simulink model "TVC_Hover_Plant_Coaxial_Articulated"  (R2025b)
settings: Solver=ode45  StartTime=0.0  StopTime=12  MaxStep=0.02  RelTol=1e-6
model workspace (MAT data in the model file):
  Sig = Simulink.Signal
  Sig.Dimensions = -1
  Sig.DimensionsMode = 'auto'
  Sig.Complexity = 'auto'
  Sig.SampleTime = -1
  Sig.SamplingMode = 'auto'
  Sig.DataType = 'auto'
  Sig1 = Simulink.Signal
  Sig1.Dimensions = -1
  Sig1.DimensionsMode = 'auto'
  Sig1.Complexity = 'auto'
  Sig1.SampleTime = -1
  Sig1.SamplingMode = 'auto'
  Sig1.DataType = 'auto'
  Sig2 = Simulink.Signal
  Sig2.Dimensions = -1
  Sig2.DimensionsMode = 'auto'
  Sig2.Complexity = 'auto'
  Sig2.SampleTime = -1
  Sig2.SamplingMode = 'auto'
  Sig2.DataType = 'auto'
  Sig3 = Simulink.Signal
  Sig3.Dimensions = -1
  Sig3.DimensionsMode = 'auto'
  Sig3.Complexity = 'auto'
  Sig3.SampleTime = -1
  Sig3.SamplingMode = 'auto'
  Sig3.DataType = 'auto'
  Sig4 = Simulink.Signal
  Sig4.Dimensions = -1
  Sig4.DimensionsMode = 'auto'
  Sig4.Complexity = 'auto'
  Sig4.SampleTime = -1
  Sig4.SamplingMode = 'auto'
  Sig4.DataType = 'auto'
  Sig5 = Simulink.Signal
  Sig5.Dimensions = -1
  Sig5.DimensionsMode = 'auto'
  Sig5.Complexity = 'auto'
  Sig5.SampleTime = -1
  Sig5.SamplingMode = 'auto'
  Sig5.DataType = 'auto'
  TVC_ARTICULATION_ENABLED = 1
  TVC_FAN1_KQ = 0.012
  TVC_FAN2_KQ = 0.012
  TVC_FAN_CG_OFFSET_M = [0; 0; 0]
  TVC_GRAVITY_MPS2 = 9.80665
  TVC_INERTIA_KGM2 = [0.003  0  0; 0  0.016  0; 0  0  0.016]
  TVC_I_FAN_CG_KGM2 = [0  0  0; 0  0  0; 0  0  0]
  TVC_I_UPPER_CG_KGM2 = [0.00105  0  0; 0  0.0056  0; 0  0  0.0056]
  TVC_JOINT_DIFF_TAU_S = 0.02
  TVC_JOINT_DIFF_TS_S = 0.01
  TVC_LINK1_M = [-0.084; 0; 0]
  TVC_LINK2_M = [-0.097; 0; 0]
  TVC_MASS_FAN_KG = 0.224
  TVC_MASS_KG = 0.8
  TVC_MASS_LINK1_KG = 0.264
  TVC_MASS_LINK2_KG = 0.248
  TVC_MASS_UPPER_KG = 0.464
  TVC_PIVOT_B_M = [-0.12; 0; 0]
  TVC_SERVO_MAX_DEG = 20
  TVC_TMAX1_N = 8
  TVC_TMAX2_N = 8
settings Model: Creator=shhan  LastModifiedBy=shhan

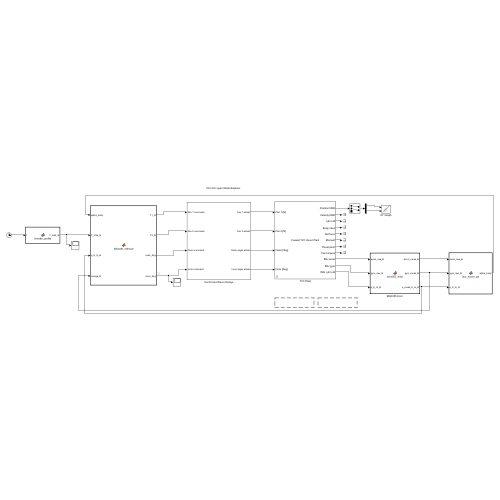
[thumbnail: Simulink's stored preview of the top-level diagram]
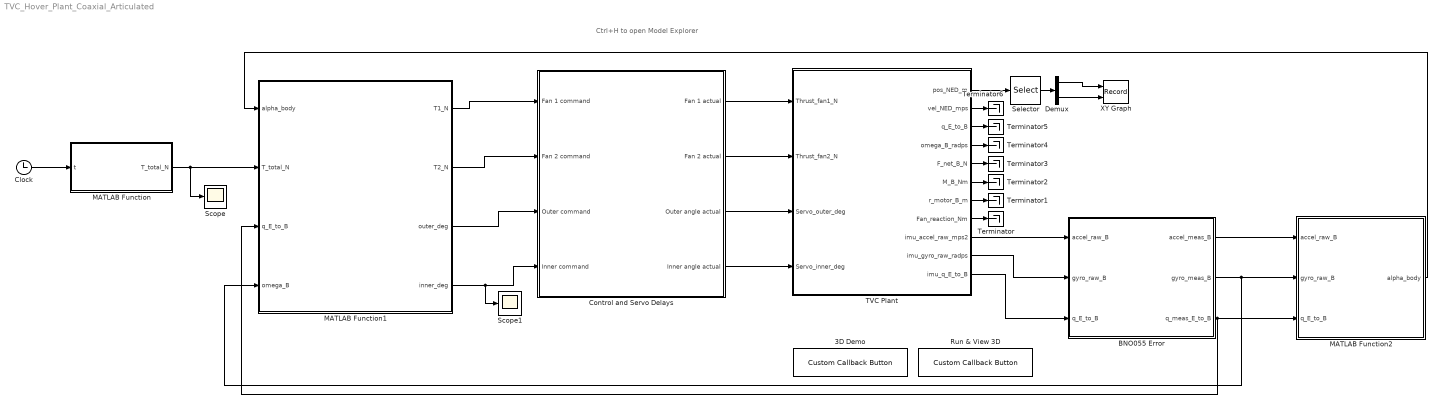
== system TVC_Hover_Plant_Coaxial_Articulated ==
  note: Ctrl+H to open Model Explorer
  3D Demo : CustomCallbackButton  Tag=TVCReplayButton  Configuration="{\"components\":[{\"name\":\"BackgroundImageComponent\",\"settings\":{\"image\":{\"size\":[0,0],\"src\":\"default\",\"srcOrientation\":\"Right\"},\"position\":[0,0,1,1]}},{\"name\":\"ButtonStateComponent\",\"settings\":{\"buttonType\":\"momentary\",\"clickFcn\":\"build_TVC_hover_plant('diagram-demo', bdroot());\",\"onValue\":1,\"position\":[0,0,1,1],\"pressDelay\":\"500\",\"pressFcn\":\"\",\"repeatInterval\":\"0\",\"states\":[{\"horizontalAlignment\":\"center\",\"image\":{\"position\":[0,0,1,1],\"size\":[1,1],\"src\":\"default\",\"srcOrientation\":\"Right\"},\"label\":{\"color\":[0.01176470588,0.01176470588,0.01176470588,1],\"icon\":{\"size\":[0,0],\"src\":\"default\",\"srcOrientation\":\"Right\"},\"iconOffset\":0,\"iconPlacement\":\"left\",\"opacity\":1,\"show\":true,\"text\":{\"content\":\"3D Demo\",\"font\":\"Helvetica\"}},\"labelOffset\":[0,0],\"verticalAlignment\":\"middle\"},{\"horizontalAlignment\":\"center\",\"image\":{\"position\":[0,0,1,1],\"size\":[1,1],\"src\":\"default\",\"srcOrientation\":\"Right\"},\"label\":{\"color\":[0.01176470588,0.01176470588,0.01176470588,1],\"icon\":{\"size\":[0,0],\"src\":\"default\",\"srcOrientation\":\"Right\"},\"iconOffset\":0,\"iconPlacement\":\"left\",\"opacity\":1,\"show\":true,\"text\":{\"content\":\"3D Demo\",\"font\":\"Helvetica\"}},\"labelOffset\":[0,0],\"verticalAlignment\":\"middle\"},{\"horizontalAlignment\":\"center\",\"image\":{\"position\":[0,0,1,1],\"size\":[1,1],\"src\":\"default\",\"srcOrientation\":\"Right\"},\"label\":{\"color\":[0.01176470588,0.01176470588,0.01176470588,1],\"icon\":{\"size\":[0,0],\"src\":\"default\",\"srcOrientation\":\"Right\"},\"iconOffset\":0,\"iconPlacement\":\"left\",\"opacity\":1,\"show\":true,\"text\":{\"content\":\"3D Demo\",\"font\":\"Helvetica\"}},\"labelOffset\":[0,0],\"verticalAlignment\":\"middle\"},{\"horizontalAlignment\":\"center\",\"image\":{\"position\":[0,0,1,1],\"size\":[1,1],\"src\":\"default\",\"srcOrientation\":\"Right\"},\"label\":{\"color\":[0.01176470588,0.01176470588,0.01176470588,1],\"icon\":{\"size\":[0,0],\"src\":\"default\",\"srcOrientation\":\"Right\"},\"iconOffset\":0,\"iconPlacement\":\"left\",\"opacity\":1,\"show\":true,\"text\":{\"content\":\"3D Demo\",\"font\":\"Helvetica\"}},\"labelOffset\":[0,0],\"verticalAlignment\":\"middle\"}]}},{\"name\":\"ForegroundImageComponent\",\"settings\":{\"image\":{\"size\":[0,0],\"src\":\"default\",\"srcOrientation\":\"Right\"},\"isForeground\":1,\"position\":[0,0,1,1]}}],\"derived\":{\"blockParameters\":{\"AutoActivate\":true,\"ButtonText\":\"3D Demo\",\"ButtonType\":\"Momentary\",\"ClickFcn\":\"build_TVC_hover_plant('diagram-demo', bdroot());\",\"OnValue\":1,\"PressDelay\":\"500\",\"PressFcn\":\"\",\"RepeatInterval\":\"0\",\"fixedAspectRatio\":\"off\"}},\"settings\":{\"BindingType\":\"standalone\",\"autoActivate\":true,\"backgroundColor\":[244,244,244,1],\"backgroundOffset\":0.2,\"backgroundOpacity\":1,\"fixedAspectRatio\":\"off\",\"foregroundColor\":[0.01176470588,0.01176470588,0.01176470588,1],\"migratedFromLegacy\":true,\"useBackgroundColor\":true,\"variant\":\"callback\",\"version\":\"R2025a\"},\"type\":\"Button\"}"  CustomBackgroundColor="{\"color\":[0.9568627451,0.9568627451,0.9568627451],\"show\":true}"
  BNO055 Error : MATLAB Function  TreatAsAtomicUnit=on
  Clock : Clock
  Control and Servo Delays : Subsystem  Tag=TVCControllerAndServoTiming
  Demux : Demux  Outputs=2
  MATLAB Function : MATLAB Function  TreatAsAtomicUnit=on
  MATLAB Function1 : MATLAB Function  TreatAsAtomicUnit=on
  MATLAB Function2 : MATLAB Function  TreatAsAtomicUnit=on
  Run & View 3D : CustomCallbackButton  Tag=TVCReplayButton  Configuration="{\"components\":[{\"name\":\"BackgroundImageComponent\",\"settings\":{\"image\":{\"size\":[0,0],\"src\":\"default\",\"srcOrientation\":\"Right\"},\"position\":[0,0,1,1]}},{\"name\":\"ButtonStateComponent\",\"settings\":{\"buttonType\":\"momentary\",\"clickFcn\":\"build_TVC_hover_plant('diagram-run', bdroot());\",\"onValue\":1,\"position\":[0,0,1,1],\"pressDelay\":\"500\",\"pressFcn\":\"\",\"repeatInterval\":\"0\",\"states\":[{\"horizontalAlignment\":\"center\",\"image\":{\"position\":[0,0,1,1],\"size\":[1,1],\"src\":\"default\",\"srcOrientation\":\"Right\"},\"label\":{\"color\":[0.01176470588,0.01176470588,0.01176470588,1],\"icon\":{\"size\":[0,0],\"src\":\"default\",\"srcOrientation\":\"Right\"},\"iconOffset\":0,\"iconPlacement\":\"left\",\"opacity\":1,\"show\":true,\"text\":{\"content\":\"Run & View 3D\",\"font\":\"Helvetica\"}},\"labelOffset\":[0,0],\"verticalAlignment\":\"middle\"},{\"horizontalAlignment\":\"center\",\"image\":{\"position\":[0,0,1,1],\"size\":[1,1],\"src\":\"default\",\"srcOrientation\":\"Right\"},\"label\":{\"color\":[0.01176470588,0.01176470588,0.01176470588,1],\"icon\":{\"size\":[0,0],\"src\":\"default\",\"srcOrientation\":\"Right\"},\"iconOffset\":0,\"iconPlacement\":\"left\",\"opacity\":1,\"show\":true,\"text\":{\"content\":\"Run & View 3D\",\"font\":\"Helvetica\"}},\"labelOffset\":[0,0],\"verticalAlignment\":\"middle\"},{\"horizontalAlignment\":\"center\",\"image\":{\"position\":[0,0,1,1],\"size\":[1,1],\"src\":\"default\",\"srcOrientation\":\"Right\"},\"label\":{\"color\":[0.01176470588,0.01176470588,0.01176470588,1],\"icon\":{\"size\":[0,0],\"src\":\"default\",\"srcOrientation\":\"Right\"},\"iconOffset\":0,\"iconPlacement\":\"left\",\"opacity\":1,\"show\":true,\"text\":{\"content\":\"Run & View 3D\",\"font\":\"Helvetica\"}},\"labelOffset\":[0,0],\"verticalAlignment\":\"middle\"},{\"horizontalAlignment\":\"center\",\"image\":{\"position\":[0,0,1,1],\"size\":[1,1],\"src\":\"default\",\"srcOrientation\":\"Right\"},\"label\":{\"color\":[0.01176470588,0.01176470588,0.01176470588,1],\"icon\":{\"size\":[0,0],\"src\":\"default\",\"srcOrientation\":\"Right\"},\"iconOffset\":0,\"iconPlacement\":\"left\",\"opacity\":1,\"show\":true,\"text\":{\"content\":\"Run & View 3D\",\"font\":\"Helvetica\"}},\"labelOffset\":[0,0],\"verticalAlignment\":\"middle\"}]}},{\"name\":\"ForegroundImageComponent\",\"settings\":{\"image\":{\"size\":[0,0],\"src\":\"default\",\"srcOrientation\":\"Right\"},\"isForeground\":1,\"position\":[0,0,1,1]}}],\"derived\":{\"blockParameters\":{\"AutoActivate\":true,\"ButtonText\":\"Run & View 3D\",\"ButtonType\":\"Momentary\",\"ClickFcn\":\"build_TVC_hover_plant('diagram-run', bdroot());\",\"OnValue\":1,\"PressDelay\":\"500\",\"PressFcn\":\"\",\"RepeatInterval\":\"0\",\"fixedAspectRatio\":\"off\"}},\"settings\":{\"BindingType\":\"standalone\",\"autoActivate\":true,\"backgroundColor\":[244,244,244,1],\"backgroundOffset\":0.2,\"backgroundOpacity\":1,\"fixedAspectRatio\":\"off\",\"foregroundColor\":[0.01176470588,0.01176470588,0.01176470588,1],\"migratedFromLegacy\":true,\"useBackgroundColor\":true,\"variant\":\"callback\",\"version\":\"R2025a\"},\"type\":\"Button\"}"  CustomBackgroundColor="{\"color\":[0.9568627451,0.9568627451,0.9568627451],\"show\":true}"
  Scope : Scope
      settings: ActiveDisplayYMinimum=-4.2053320985847265  ActiveDisplayYMaximum=11.307950061200437
  Scope1 : Scope
      settings: DataLoggingVariableName=ScopeData2
  Selector : Selector  InputPortWidth=3  IndexOptions=Index vector (dialog)  Indices=[1 2]  OutputSizes=1
  TVC Plant : Subsystem  mask{mass_kg=TVC_MASS_UPPER_KG + TVC_MASS_LINK1_KG + TVC_MASS_LINK2_KG + TVC_MASS_FAN_KG, inertia_kgm2=TVC_INERTIA_KGM2, g_mps2=TVC_GRAVITY_MPS2, pivot_B_m=TVC_PIVOT_B_M, link1_m=TVC_LINK1_M, link2_m=TVC_LINK2_M, fan1_kq=TVC_FAN1_KQ, fan2_kq=TVC_FAN2_KQ, pos0_NED_m=[0 0 0], vel0_B_mps=[0 0 0], eul0_rad=[0 pi/2 0], omega0_B_radps=[0 0 0]}
      mask prompts: mass_kg "Mass (kg)"; inertia_kgm2 "Inertia at center of mass (kg m^2)"; g_mps2 "Gravity (m/s^2)"; pivot_B_m "Center of mass to outer joint in body axes (m)"; link1_m "Outer to inner joint in outer link axes (m)"; link2_m "Inner joint to thrust point in inner link axes (m)"; fan1_kq "Fan 1 torque per unit thrust (N*m/N)"; fan2_kq "Fan 2 torque per unit thrust (N*m/N)"; pos0_NED_m "Initial position in NED (m)"; vel0_B_mps "Initial velocity in body axes (m/s)"; eul0_rad "Initial [roll pitch yaw] (rad)"; omega0_B_radps "Initial body angular rates (rad/s)"
      mask help: Two coaxial counter-rotating fans on a serial two-joint TVC. At zero joint angles, thrust points along body +X. Joint angles are in degrees. Position and velocity use NED axes.
      mask Help: Enter link vectors in their own neutral joint frames. The pivot vector starts at the fixed center of mass and ends at the outer servo axis. The first link ends at the inner servo axis. The second link ends at the thrust application point. Inertia is about the center of mass. The model uses actual joint angles as inputs and fixed mass properties. Enter nonnegative torque gains in N*m/N. Fan 1 applies negative and fan 2 applies positive reaction torque along the common thrust axis.
      mask Display:
      | disp('Coaxial TVC Hover Plant');
      | port_label('input', 1, 'Fan 1 [N]');
      | port_label('input', 2, 'Fan 2 [N]');
      | port_label('input', 3, 'Outer [deg]');
      | port_label('input', 4, 'Inner [deg]');
      | port_label('output', 1, 'Position NED');
      | port_label('output', 2, 'Velocity NED');
      | port_label('output', 3, 'q E to B');
      | port_label('output', 4, 'Body rates');
      | port_label('output', 5, 'Net force');
      | port_label('output', 6, 'Moment');
      | port_label('output', 7, 'Thrust point');
      | port_label('output', 8, 'Fan torques');
      | port_label('output', 9, 'IMU accel');
      | port_label('output', 10, 'IMU gyro');
      | port_label('output', 11, 'IMU q E to B');
  Terminator{,1..6} (7 alike) : Terminator
  XY Graph : Record  NumPorts=2.0  FileSettingsInternal="{\"entries\":[{\"content\":{\"excelSettings\":{\"content\":{},\"type\":\"Streamout.ExcelSettings\"},\"parquetSettings\":{\"content\":{},\"type\":\"Streamout.ParquetSettings\"}},\"type\":\"Streamout.FileSettingStorage\",\"uuid\":\"\"}],\"packageUris\":[\"http:\\/\\/schema.mathworks.com\\/mf0\\/streamout_blocks\\/R2020a\"],\"version\":\"1.0\"}"  FrameSettings=[0, 0]  Layout=[1 1]  SignalsInternal="{\"entries\":[{\"content\":{\"signals\":[{\"content\":{\"blockPath\":[],\"dimensions\":[1],\"domain\":\"\",\"lineColor\":\"#a2142f\",\"plots\":[ 1 ],\"port\":1,\"sid\":[\"\"],\"signalID\":1,\"signalName\":\"Demux:1\"},\"type\":\"RecordBlkView.Signal\",\"uuid\":\"\"},{\"content\":{\"blockPath\":[],\"dimensions\":[1],\"domain\":\"\",\"lineColor\":\"#139fff\",\"plots\":[ 1 ],\"port\":2,\"sid\":[\"\"],\"signalID\":2,\"signalName\":\"Demux:2\"},\"type\":\"RecordBlkView.Signal\",\"uuid\":\"\"}]},\"type\":\"RecordBlkView.InputSignals\",\"uuid\":\"\"}],\"packageUris\":[\"http:\\/\\/schema.mathworks.com\\/mf0\\/streamout_blocks\\/R2020a\"],\"version\":\"1.0\"}"  VisualizationBindings="{\"xyplotplugin\":{\"info\":[{\"series\":[{\"bindingParametersList\":[{\"parameter\":\"X-Axis\",\"signalID\":2,\"signalName\":\"Demux:2\"},{\"parameter\":\"Y-Axis\",\"signalID\":1,\"signalName\":\"Demux:1\"}],\"seriesID\":0}],\"subplotID\":1}]}}"  CompatibilityTag=XY
  wires:
  TVC Plant/10(imu_gyro_raw_radps) -> BNO055 Error/2(gyro_raw_B)
  TVC Plant/11(imu_q_E_to_B) -> BNO055 Error/3(q_E_to_B)
  MATLAB Function2/1(alpha_body) -> MATLAB Function1/1(alpha_body)
  MATLAB Function/1(T_total_N) -> Scope/1, MATLAB Function1/2(T_total_N)
  Clock/1 -> MATLAB Function/1(t)
  TVC Plant/9(imu_accel_raw_mps2) -> BNO055 Error/1(accel_raw_B)
  BNO055 Error/3(q_meas_E_to_B) -> MATLAB Function1/3(q_E_to_B), MATLAB Function2/3(q_E_to_B)
  BNO055 Error/2(gyro_meas_B) -> MATLAB Function1/4(omega_B), MATLAB Function2/2(gyro_raw_B)
  BNO055 Error/1(accel_meas_B) -> MATLAB Function2/1(accel_raw_B)
  MATLAB Function1/1(T1_N) -> Control and Servo Delays/1(Fan 1 command)
  Control and Servo Delays/1(Fan 1 actual) -> TVC Plant/1(Thrust_fan1_N)
  MATLAB Function1/2(T2_N) -> Control and Servo Delays/2(Fan 2 command)
  Control and Servo Delays/2(Fan 2 actual) -> TVC Plant/2(Thrust_fan2_N)
  MATLAB Function1/3(outer_deg) -> Control and Servo Delays/3(Outer command)
  Control and Servo Delays/3(Outer angle actual) -> TVC Plant/3(Servo_outer_deg)
  MATLAB Function1/4(inner_deg) -> Scope1/1, Control and Servo Delays/4(Inner command)
  Control and Servo Delays/4(Inner angle actual) -> TVC Plant/4(Servo_inner_deg)
  TVC Plant/8(Fan_reaction_Nm) -> Terminator/1
  TVC Plant/7(r_motor_B_m) -> Terminator1/1
  TVC Plant/6(M_B_Nm) -> Terminator2/1
  TVC Plant/5(F_net_B_N) -> Terminator3/1
  TVC Plant/4(omega_B_radps) -> Terminator4/1
  TVC Plant/3(q_E_to_B) -> Terminator5/1
  TVC Plant/2(vel_NED_mps) -> Terminator6/1
  TVC Plant/1(pos_NED_m) -> Selector/1
  Selector/1 -> Demux/1
  Demux/2 -> XY Graph/2
  Demux/1 -> XY Graph/1

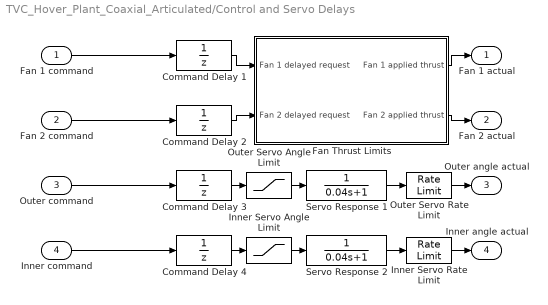
== system TVC_Hover_Plant_Coaxial_Articulated/Control and Servo Delays ==
  Fan 1 command : Inport
  Fan 2 command : Inport  Port=2
  Outer command : Inport  Port=3
  Inner command : Inport  Port=4
  Command Delay {1..4} (4 alike) : UnitDelay  SampleTime=0.01  HasFrameUpgradeWarning=on
  Fan Thrust Limits : Subsystem  Tag=TVCFanThrustLimits
  Inner Servo Angle Limit : Saturate  Tag=TVCMG996RLimit  UpperLimit=min(20,TVC_SERVO_MAX_DEG)  LowerLimit=-(min(20,TVC_SERVO_MAX_DEG))
  Inner Servo Rate Limit : RateLimiter  Tag=TVCMG996RLimit  RisingSlewLimit=400  FallingSlewLimit=-400
  Outer Servo Angle Limit : Saturate  Tag=TVCMG996RLimit  UpperLimit=min(20,TVC_SERVO_MAX_DEG)  LowerLimit=-(min(20,TVC_SERVO_MAX_DEG))
  Outer Servo Rate Limit : RateLimiter  Tag=TVCMG996RLimit  RisingSlewLimit=400  FallingSlewLimit=-400
  Servo Response 1 : TransferFcn  Numerator=1  Denominator=[0.04 1]
  Servo Response 2 : TransferFcn  Numerator=1  Denominator=[0.04 1]
  Fan 1 actual : Outport
  Fan 2 actual : Outport  Port=2
  Outer angle actual : Outport  Port=3
  Inner angle actual : Outport  Port=4
  wires:
  Fan 1 command/1 -> Command Delay 1/1
  Fan 2 command/1 -> Command Delay 2/1
  Outer command/1 -> Command Delay 3/1
  Inner command/1 -> Command Delay 4/1
  Command Delay 1/1 -> Fan Thrust Limits/1(Fan 1 delayed request)
  Fan Thrust Limits/1(Fan 1 applied thrust) -> Fan 1 actual/1
  Command Delay 2/1 -> Fan Thrust Limits/2(Fan 2 delayed request)
  Fan Thrust Limits/2(Fan 2 applied thrust) -> Fan 2 actual/1
  Command Delay 3/1 -> Outer Servo Angle Limit/1
  Outer Servo Angle Limit/1 -> Servo Response 1/1
  Servo Response 1/1 -> Outer Servo Rate Limit/1
  Outer Servo Rate Limit/1 -> Outer angle actual/1
  Command Delay 4/1 -> Inner Servo Angle Limit/1
  Inner Servo Angle Limit/1 -> Servo Response 2/1
  Servo Response 2/1 -> Inner Servo Rate Limit/1
  Inner Servo Rate Limit/1 -> Inner angle actual/1

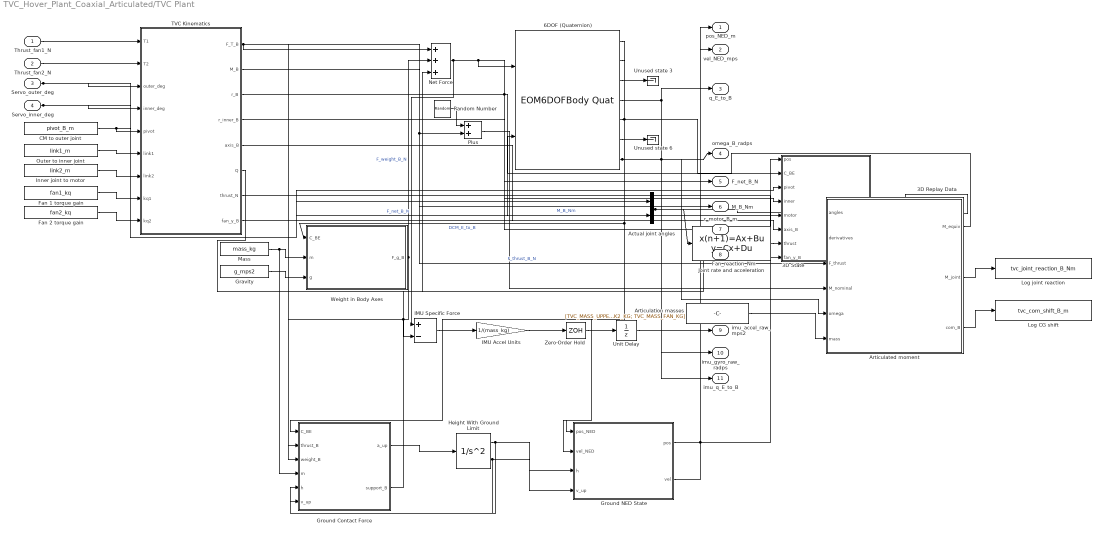
== system TVC_Hover_Plant_Coaxial_Articulated/TVC Plant ==
  Thrust_fan1_N : Inport  OutDataTypeStr=double  PortDimensions=1
  Thrust_fan2_N : Inport  Port=2  OutDataTypeStr=double  PortDimensions=1
  Servo_outer_deg : Inport  Port=3  OutDataTypeStr=double  PortDimensions=1
  Servo_inner_deg : Inport  Port=4  OutDataTypeStr=double  PortDimensions=1
  3D Replay Data : ToWorkspace  VariableName=TVC3D  SaveFormat=Timeseries  SampleTime=-1
  3D State : MATLAB Function  TreatAsAtomicUnit=on
  6DOF (Quaternion) : EOM6DOFBodyQuat  xme_0=pos0_NED_m  Vm_0=vel0_B_mps  eul_0=eul0_rad  pm_0=omega0_B_radps  mass_0=mass_kg  inertia=inertia_kgm2
  Actual joint angles : Mux  Inputs=2
  Articulated moment : MATLAB Function  TreatAsAtomicUnit=on
  Articulation masses : Constant  Value=[TVC_MASS_UPPER_KG; TVC_MASS_LINK1_KG; TVC_MASS_LINK2_KG; TVC_MASS_FAN_KG]
  CM to outer joint : Constant  Value=pivot_B_m
  Fan 1 torque gain : Constant  Value=fan1_kq
  Fan 2 torque gain : Constant  Value=fan2_kq
  Gravity : Constant  Value=g_mps2
  Ground Contact Force : MATLAB Function  TreatAsAtomicUnit=on
  Ground NED State : MATLAB Function  TreatAsAtomicUnit=on
  Height With Ground Limit : SecondOrderIntegrator  ICX=max(0, -pos0_NED_m(3))  LimitX=on  LowerLimitX=0  ICDXDT=sin(eul0_rad(2))*vel0_B_mps(1)-cos(eul0_rad(2))*(sin(eul0_rad(1))*vel0_B_mps(2)+cos(eul0_rad(1))*vel0_B_mps(3))
  IMU Accel Units : Gain  Gain=1/(mass_kg)
  IMU Specific Force : Sum  Inputs=+-
  Inner joint to motor : Constant  Value=link2_m
  Joint rate and acceleration : DiscreteStateSpace  A=[zeros(2,6);-((1-(exp(-TVC_JOINT_DIFF_TS_S/TVC_JOINT_DIFF_TAU_S)))/TVC_JOINT_DIFF_TS_S)*eye(2),(exp(-TVC_JOINT_DIFF_TS_S/TVC_JOINT_DIFF_TAU_S))*eye(2),zeros(2);-((1-(exp(-TVC_JOINT_DIFF_TS_S/TVC_JOINT_DIFF_TAU_S)))/TVC_JOINT_DIFF_TS_S)^2*eye(2),((1-(exp(-TVC_JOINT_DIFF_TS_S/TVC_JOINT_DIFF_TAU_S)))/TVC_JOINT_DIFF_TS_S)*((exp(-TVC_JOINT_DIFF_TS_S/TVC_JOINT_DIFF_TAU_S))-1)*eye(2),(exp(-TVC_JOINT_DIFF_TS_S/TVC_JOINT_DIFF_TAU_S))*eye(2)]  B=[eye(2);((1-(exp(-TVC_JOINT_DIFF_TS_S/TVC_JOINT_DIFF_TAU_S)))/TVC_JOINT_DIFF_TS_S)*eye(2);((1-(exp(-TVC_JOINT_DIFF_TS_S/TVC_JOINT_DIFF_TAU_S)))/TVC_JOINT_DIFF_TS_S)^2*eye(2)]  C=[-((1-(exp(-TVC_JOINT_DIFF_TS_S/TVC_JOINT_DIFF_TAU_S)))/TVC_JOINT_DIFF_TS_S)*eye(2),(exp(-TVC_JOINT_DIFF_TS_S/TVC_JOINT_DIFF_TAU_S))*eye(2),zeros(2);-((1-(exp(-TVC_JOINT_DIFF_TS_S/TVC_JOINT_DIFF_TAU_S)))/TVC_JOINT_DIFF_TS_S)^2*eye(2),((1-(exp(-TVC_JOINT_DIFF_TS_S/TVC_JOINT_DIFF_TAU_S)))/TVC_JOINT_DIFF_TS_S)*((exp(-TVC_JOINT_DIFF_TS_S/TVC_JOINT_DIFF_TAU_S))-1)*eye(2),(exp(-TVC_JOINT_DIFF_TS_S/TVC_JOINT_DIFF_TAU_S))*eye(2)]  D=[((1-(exp(-TVC_JOINT_DIFF_TS_S/TVC_JOINT_DIFF_TAU_S)))/TVC_JOINT_DIFF_TS_S)*eye(2);((1-(exp(-TVC_JOINT_DIFF_TS_S/TVC_JOINT_DIFF_TAU_S)))/TVC_JOINT_DIFF_TS_S)^2*eye(2)]  InitialCondition=zeros(6,1)  SampleTime=TVC_JOINT_DIFF_TS_S
  Log CG shift : ToWorkspace  VariableName=tvc_com_shift_B_m  SaveFormat=Timeseries  SampleTime=-1
  Log joint reaction : ToWorkspace  VariableName=tvc_joint_reaction_B_Nm  SaveFormat=Timeseries  SampleTime=-1
  Mass : Constant  Value=mass_kg
  Net Force : Sum  Inputs=+++
  Outer to inner joint : Constant  Value=link1_m
  Plus : Sum
  Random Number : RandomNumber  Variance=0.005  SampleTime=0.01  VectorParams1D=off
  TVC Kinematics : MATLAB Function  TreatAsAtomicUnit=on
  Unit Delay : UnitDelay  InitialCondition=[g_mps2; 0; 0]  SampleTime=0.01  HasFrameUpgradeWarning=on
  Unused state 3 : Terminator
  Unused state 6 : Terminator
  Weight in Body Axes : MATLAB Function  TreatAsAtomicUnit=on
  Zero-Order Hold : ZeroOrderHold  SampleTime=0.01
  pos_NED_m : Outport
  vel_NED_mps : Outport  Port=2
  q_E_to_B : Outport  Port=3
  omega_B_radps : Outport  Port=4
  F_net_B_N : Outport  Port=5
  M_B_Nm : Outport  Port=6
  r_motor_B_m : Outport  Port=7
  Fan_reaction_Nm : Outport  Port=8
  imu_accel_raw_mps2 : Outport  Port=9
  imu_gyro_raw_radps : Outport  Port=10
  imu_q_E_to_B : Outport  Port=11
  wires:
  Thrust_fan1_N/1 -> TVC Kinematics/1(T1)
  Thrust_fan2_N/1 -> TVC Kinematics/2(T2)
  Servo_outer_deg/1 -> TVC Kinematics/3(outer_deg), Actual joint angles/1
  Servo_inner_deg/1 -> TVC Kinematics/4(inner_deg), Actual joint angles/2
  CM to outer joint/1 -> TVC Kinematics/5(pivot), 3D State/3(pivot)
  Outer to inner joint/1 -> TVC Kinematics/6(link1)
  Inner joint to motor/1 -> TVC Kinematics/7(link2)
  Fan 1 torque gain/1 -> TVC Kinematics/8(kq1)
  Fan 2 torque gain/1 -> TVC Kinematics/9(kq2)
  6DOF (Quaternion)/5 -> Ground Contact Force/1(C_BE), Weight in Body Axes/1(C_BE), 3D State/2(C_BE)  "DCM_E_to_B"
  Mass/1 -> Weight in Body Axes/2(m), Ground Contact Force/4(m)
  Gravity/1 -> Weight in Body Axes/3(g)
  TVC Kinematics/1(F_T_B) -> Net Force/1, Ground Contact Force/2(thrust_B), Articulated moment/3(F_thrust)  "F_thrust_B_N"
  Weight in Body Axes/1(F_g_B) -> IMU Specific Force/2, Ground Contact Force/3(weight_B), Net Force/2  "F_weight_B_N"
  Net Force/1 -> 6DOF (Quaternion)/1, F_net_B_N/1, IMU Specific Force/1  "F_net_B_N"
  TVC Kinematics/2(M_B) -> Plus/2, M_B_Nm/1  "M_B_Nm"
  6DOF (Quaternion)/2 -> Ground NED State/1(pos_NED)
  6DOF (Quaternion)/1 -> Ground NED State/2(vel_NED)
  6DOF (Quaternion)/4 -> q_E_to_B/1, imu_q_E_to_B/1
  6DOF (Quaternion)/7 -> omega_B_radps/1, imu_gyro_raw_radps/1, Articulated moment/5(omega)
  TVC Kinematics/3(r_B) -> r_motor_B_m/1, 3D State/5(motor)
  TVC Kinematics/6(Q) -> Fan_reaction_Nm/1
  6DOF (Quaternion)/3 -> Unused state 3/1
  6DOF (Quaternion)/6 -> Unused state 6/1
  TVC Kinematics/4(r_inner_B) -> 3D State/4(inner)
  TVC Kinematics/5(axis_B) -> 3D State/6(axis_B)
  TVC Kinematics/7(thrust_N) -> 3D State/7(thrust)
  TVC Kinematics/8(fan_y_B) -> 3D State/8(fan_y_B)
  3D State/1(frame) -> 3D Replay Data/1
  Random Number/1 -> Plus/1
  IMU Specific Force/1 -> IMU Accel Units/1
  IMU Accel Units/1 -> Zero-Order Hold/1
  Zero-Order Hold/1 -> Unit Delay/1
  Unit Delay/1 -> imu_accel_raw_mps2/1
  Height With Ground Limit/1 -> Ground Contact Force/5(h), Ground NED State/3(h)
  Height With Ground Limit/2 -> Ground Contact Force/6(v_up), Ground NED State/4(v_up)
  Ground Contact Force/1(a_up) -> Height With Ground Limit/1
  Ground Contact Force/2(support_B) -> Net Force/3
  Ground NED State/1(pos) -> pos_NED_m/1, 3D State/1(pos)
  Ground NED State/2(vel) -> vel_NED_mps/1
  Actual joint angles/1 -> Joint rate and acceleration/1, Articulated moment/1(angles)
  Joint rate and acceleration/1 -> Articulated moment/2(derivatives)
  Plus/1 -> Articulated moment/4(M_nominal)
  Articulation masses/1 -> Articulated moment/6(mass)
  Articulated moment/1(M_equiv) -> 6DOF (Quaternion)/2
  Articulated moment/2(M_joint) -> Log joint reaction/1
  Articulated moment/3(com_B) -> Log CG shift/1

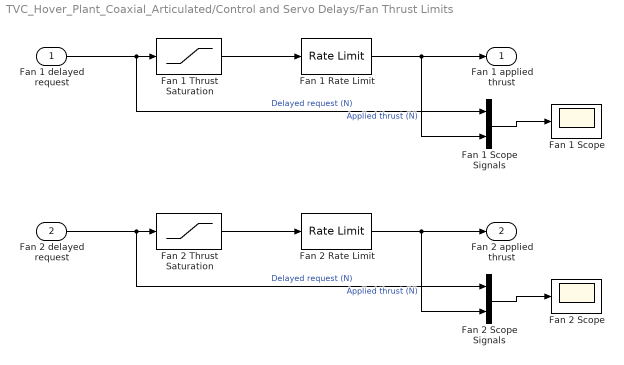
== system TVC_Hover_Plant_Coaxial_Articulated/Control and Servo Delays/Fan Thrust Limits ==
  Fan 1 delayed request : Inport
  Fan 2 delayed request : Inport  Port=2
  Fan 1 Rate Limit : RateLimiter  RisingSlewLimit=30  FallingSlewLimit=-40  SampleTimeMode=inherited
  Fan 1 Scope : Scope
      settings: ActiveDisplayYMinimum=-4.2104178950600506  ActiveDisplayYMaximum=6.9345692292578747
  Fan 1 Scope Signals : Mux  Inputs=2
  Fan 1 Thrust Saturation : Saturate  UpperLimit=TVC_TMAX1_N  LowerLimit=0
  Fan 2 Rate Limit : RateLimiter  RisingSlewLimit=30  FallingSlewLimit=-40  SampleTimeMode=inherited
  Fan 2 Scope : Scope
      settings: ActiveDisplayYMinimum=-0.7551085161181017  ActiveDisplayYMaximum=6.7959766450629173
  Fan 2 Scope Signals : Mux  Inputs=2
  Fan 2 Thrust Saturation : Saturate  UpperLimit=TVC_TMAX2_N  LowerLimit=0
  Fan 1 applied thrust : Outport
  Fan 2 applied thrust : Outport  Port=2
  wires:
  Fan 1 delayed request/1 -> Fan 1 Thrust Saturation/1, Fan 1 Scope Signals/1  "Delayed request (N)"
  Fan 1 Thrust Saturation/1 -> Fan 1 Rate Limit/1
  Fan 1 Rate Limit/1 -> Fan 1 applied thrust/1, Fan 1 Scope Signals/2  "Applied thrust (N)"
  Fan 1 Scope Signals/1 -> Fan 1 Scope/1
  Fan 2 delayed request/1 -> Fan 2 Thrust Saturation/1, Fan 2 Scope Signals/1  "Delayed request (N)"
  Fan 2 Thrust Saturation/1 -> Fan 2 Rate Limit/1
  Fan 2 Rate Limit/1 -> Fan 2 applied thrust/1, Fan 2 Scope Signals/2  "Applied thrust (N)"
  Fan 2 Scope Signals/1 -> Fan 2 Scope/1

== matlab function TVC_Hover_Plant_Coaxial_Articulated/TVC Plant/Ground Contact Force ==
  data: C_BE input; a_up output; thrust_B input; weight_B input; m input; h input; v_up input; support_B output
function [a_up, support_B] = contact(C_BE, thrust_B, weight_B, m, h, v_up)
%#codegen
up_B = -C_BE(:,3);
a_up = dot(up_B, thrust_B(:) + weight_B(:))/m;
support_B = zeros(3,1);
if h <= 0 && v_up <= 0
    support_B = max(0, -m*a_up)*up_B;
end
end

== matlab function TVC_Hover_Plant_Coaxial_Articulated/MATLAB Function2 ==
  settings: updateMethod=DISCRETE  sampleTime=0.01
  data: accel_raw_B input; alpha_body output; gyro_raw_B input; q_E_to_B input; TVC_GRAVITY_MPS2 parameter double size=[1 1]
function alpha_body = imu_hover_pd(accel_raw_B, gyro_raw_B, q_E_to_B, ...
    TVC_GRAVITY_MPS2)
%#codegen
% accel_raw_B: 동체 기준 가속도계 비력 [m/s^2]
% gyro_raw_B : 동체 기준 각속도 [rad/s]
% q_E_to_B   : 6DOF 쿼터니언 [w; x; y; z]
% alpha_body : 동체 기준 목표 각가속도 [rad/s^2]

%% 설정값
Ts = 0.01;                   % 블록 Sample time과 동일하게 [s]
g = TVC_GRAVITY_MPS2;
v_ref_NED = [0; 0; 0];        % [North; East; Down] [m/s]

K_vel = [47.5; 51.5];               % [North; East] 속도 오차 게인
K_acc = [0.3; 0.0];               % [North; East] 가속도 감쇠 게인
tau_acc = 0.060;               % 감쇠에 쓰는 가속도 필터 시정수 [s]
tilt_max_deg = 8.0;

Kp_att = 69.2;
Kd_att = 24.1;
q_base = [sqrt(2)/2; 0; sqrt(2)/2; 0];

persistent v_est a_filt q_prev gyro_prev
if isempty(v_est)
    v_est = zeros(3, 1);      % 정지 상태에서 시작한다고 가정
    a_filt = zeros(3, 1);
    q_prev = [sqrt(2)/2; 0; sqrt(2)/2; 0];
    gyro_prev = zeros(3, 1);
end

%% 1. 저장된 속도와 가속도로 목표 자세 계산
v_err = v_ref_NED - v_est;
tilt_NE = K_vel .* v_err(1:2) - K_acc .* a_filt(1:2);
requested_deg = norm(tilt_NE);

q_target = q_base;
if requested_deg > 1e-9
    half_angle = min(requested_deg, tilt_max_deg) * pi/360;
    axis_E = [tilt_NE(2); -tilt_NE(1); 0] / requested_deg;
    q_tilt = [cos(half_angle); sin(half_angle)*axis_E];
    q_target = quat_mul(q_tilt, q_base);
end

%% 2. 쿼터니언 자세 PD로 목표 각가속도 계산
q_err = quat_mul([q_prev(1); -q_prev(2:4)], q_target);

if q_err(1) < 0
    q_err = -q_err;
end

v_err_q = q_err(2:4);
s = norm(v_err_q);
if s < 1e-8
    e_body = 2*v_err_q;
else
    e_body = (2*atan2(s, q_err(1))/s) * v_err_q;
end

alpha_body = Kp_att*e_body - Kd_att*gyro_prev;

%% 3. 현재 IMU 입력으로 다음 샘플의 상태 갱신
q = q_E_to_B(:);
q_norm = norm(q);

if isfinite(q_norm) && q_norm > 1e-12
    q = q/q_norm;
    f_B = accel_raw_B(:);
    u = q(2:4);

    % Body -> NED 벡터 회전
    f_NED = f_B + 2*cross(u, cross(u, f_B) + q(1)*f_B);
    a_NED = f_NED + [0; 0; g];

    v_est = v_est + Ts*a_NED;

    beta = 1 - exp(-Ts/tau_acc);
    a_filt = a_filt + beta*(a_NED - a_filt);
    q_prev = q;
end

gyro_prev = gyro_raw_B(:);
end

function q = quat_mul(p, r)
q = [p(1)*r(1) - dot(p(2:4), r(2:4));
     p(1)*r(2:4) + r(1)*p(2:4) + cross(p(2:4), r(2:4))];
end

== matlab function TVC_Hover_Plant_Coaxial_Articulated/TVC Plant/Ground NED State ==
  data: pos_NED input; pos output; vel_NED input; h input; v_up input; vel output
function [pos, vel] = with_ground(pos_NED, vel_NED, h, v_up)
%#codegen
pos = [pos_NED(1); pos_NED(2); -h];
vel = [vel_NED(1); vel_NED(2); -v_up];
end

== matlab function TVC_Hover_Plant_Coaxial_Articulated/BNO055 Error ==
  settings: updateMethod=DISCRETE  sampleTime=0.01
  data: accel_raw_B input; accel_meas_B output; gyro_raw_B input; q_E_to_B input; gyro_meas_B output; q_meas_E_to_B output; TVC_GRAVITY_MPS2 parameter double size=[1 1]
function [accel_meas_B, gyro_meas_B, q_meas_E_to_B] = ...
    bno055_error(accel_raw_B, gyro_raw_B, q_E_to_B, ...
    TVC_GRAVITY_MPS2)
%#codegen
% 입력과 출력 단위: 가속도 m/s^2, 자이로 rad/s
% 쿼터니언: Earth -> Body, [w; x; y; z]

Ts = 0.01;                          % 블록의 Sample time과 동일하게
g = TVC_GRAVITY_MPS2;
rad = pi/180;

% Bosch 전형값. 가속도계 유효 대역폭은 47 Hz로 가정
sigma_accel = 150e-6 * g * sqrt(47);
sigma_gyro  = 0.10 * rad;

% 레지스터 출력 분해능
accel_lsb = 0.01;                   % m/s^2 모드
gyro_lsb  = rad/16;                 % °/s 모드를 rad/s로 변환
quat_lsb  = 2^-14;

% 선택적 오차 시험
bias_scale  = 0.0;                  % 1이면 ±80 mg, ±1 °/s 범위
sigma_q_deg = 0.0;                  % 예: 0.3이면 축당 0.3° RMS 가정
tau_q       = 0.30;                 % 자세 오차가 변하는 시정수 [s]

persistent bias_accel bias_gyro theta initialized
if isempty(initialized)
    bias_accel = zeros(3, 1);
    bias_gyro  = zeros(3, 1);
    theta      = zeros(3, 1);
    initialized = false;
end

% 바이어스는 시뮬레이션 시작 시 축별로 한 번 뽑아 유지
if ~initialized
    if bias_scale > 0
        bias_accel = bias_scale * (80e-3*g) * (2*rand(3, 1) - 1);
        bias_gyro  = bias_scale * rad       * (2*rand(3, 1) - 1);
    end
    initialized = true;
end

a = accel_raw_B(:) + bias_accel + sigma_accel*randn(3, 1);
w = gyro_raw_B(:)  + bias_gyro  + sigma_gyro*randn(3, 1);

accel_meas_B = accel_lsb * round(a/accel_lsb);
gyro_meas_B  = gyro_lsb  * round(w/gyro_lsb);

q = q_E_to_B(:);
q = q/norm(q);

if sigma_q_deg > 0
    rho = exp(-Ts/tau_q);
    theta = rho*theta + sqrt(1-rho^2)*(sigma_q_deg*rad)*randn(3, 1);

    angle = norm(theta);
    if angle > 1e-12
        u = sin(angle/2)*theta/angle;
        c = cos(angle/2);
        v = q(2:4);

        % 동체 축 기준의 작은 자세 오차를 합성
        q = [q(1)*c - dot(v, u);
             q(1)*u + c*v + cross(v, u)];
    end
end

q = quat_lsb * round(q/quat_lsb);
q_meas_E_to_B = q/norm(q);
end

== matlab function TVC_Hover_Plant_Coaxial_Articulated/TVC Plant/Articulated moment ==
  data: angles input; M_equiv output; derivatives input; F_thrust input; M_nominal input; omega input; mass input; M_joint output; com_B output; TVC_PIVOT_B_M parameter double size=[3 1]; TVC_LINK1_M parameter double size=[3 1]; TVC_LINK2_M parameter double size=[3 1]; TVC_INERTIA_KGM2 parameter double size=[3 3]; TVC_I_UPPER_CG_KGM2 parameter double size=[3 3]; TVC_I_FAN_CG_KGM2 parameter double size=[3 3]; TVC_FAN_CG_OFFSET_M parameter double size=[3 1]; TVC_ARTICULATION_ENABLED parameter double size=[1 1]
function [M_equiv, M_joint, com_B] = articulatedMoment(angles, derivatives, F_thrust, ...
    M_nominal, omega, mass, TVC_PIVOT_B_M, TVC_LINK1_M, TVC_LINK2_M, ...
TVC_INERTIA_KGM2, TVC_I_UPPER_CG_KGM2, TVC_I_FAN_CG_KGM2, ...
TVC_FAN_CG_OFFSET_M, TVC_ARTICULATION_ENABLED)
%#codegen
% All vectors are expressed in the upper body's axes. Its origin is the
% neutral total CG. The 6DOF translation states track the instantaneous CG.
% Joint motion is prescribed by the existing servo dynamics. This solves
% the upper attitude by total angular momentum balance about the total CG.

M_equiv = M_nominal(:);
M_joint = zeros(3,1);
com_B = zeros(3,1);
if TVC_ARTICULATION_ENABLED == 0
    return
end

m = mass(:);
assert(all(isfinite(m)) && m(1) > 0 && all(m(2:4) >= 0));
total = sum(m);
p = TVC_PIVOT_B_M(:);
d1 = TVC_LINK1_M(:);
d2 = TVC_LINK2_M(:);
dF = d2 + TVC_FAN_CG_OFFSET_M(:);
E = eye(3);

% Infer the fixed upper CG from the measured neutral total CG (r = 0).
upperCG = -(m(2)*(p+d1/2) + m(3)*(p+d1+d2/2) + m(4)*(p+d1+dF))/m(1);
angles = (pi/180)*angles(:);
rates = (pi/180)*derivatives(1:2);
accel = (pi/180)*derivatives(3:4);
c1 = cos(angles(1)); s1 = sin(angles(1));
c2 = cos(angles(2)); s2 = sin(angles(2));
R1 = [c1 0 s1; 0 1 0; -s1 0 c1];
R12 = R1*[c2 -s2 0; s2 c2 0; 0 0 1];
y = [0;1;0];
z = R1(:,3);
u1 = rates(1)*y;
ud1 = accel(1)*y;
u12 = u1 + rates(2)*z;
ud12 = ud1 + accel(2)*z + rates(2)*cross(u1,z);

l1 = R1*d1;
l2cg = R12*(d2/2);
lf = R12*dF;
[v1, a1] = pointDerivatives(l1, u1, ud1);
[v2, a2] = pointDerivatives(l2cg, u12, ud12);
[vf, af] = pointDerivatives(lf, u12, ud12);
origin = zeros(3,1);
locations = [upperCG, p+l1/2, p+l1+l2cg, p+l1+lf];
velocities = [origin, v1/2, v1+v2, v1+vf];
accelerations = [origin, a1/2, a1+a2, a1+af];
com_B = locations*m/total;
comRate = velocities*m/total;
comAccel = accelerations*m/total;

rotations = [origin, u1, u12, u12];
rotationRates = [origin, ud1, ud12, ud12];
intrinsic = cat(3, TVC_I_UPPER_CG_KGM2, rodTensor(m(2), l1), ...
    rodTensor(m(3), R12*d2), R12*TVC_I_FAN_CG_KGM2*R12.');
J = zeros(3);
Jrate = zeros(3);
h = zeros(3,1);
hRate = zeros(3,1);
for k = 1:4
    r = locations(:,k)-com_B;
    v = velocities(:,k)-comRate;
    a = accelerations(:,k)-comAccel;
    I = intrinsic(:,:,k);
    u = rotations(:,k);
    S = skew(u);
    IRate = S*I - I*S;
    J = J + I + m(k)*(dot(r,r)*E - r*r.');
    Jrate = Jrate + IRate + m(k)*(2*dot(r,v)*E - v*r.' - r*v.');
    h = h + I*u + m(k)*cross(r,v);
    hRate = hRate + IRate*u + I*rotationRates(:,k) + m(k)*cross(r,a);
end

w = omega(:);
% H = J*w + h. Apply inertial Euler balance dH_B/dt + w x H = M_external.
% Existing thrust moment is about the neutral CG; translate it to the new CG.
M_about_CG = M_nominal(:) - cross(com_B, F_thrust(:));
M_joint = -hRate - cross(w,h);
alpha = J \ (M_about_CG + M_joint - Jrate*w - cross(w,J*w));
Jref = TVC_INERTIA_KGM2;
% The carrier is a fixed-inertia 6DOF. Feed the moment that gives this alpha.
M_equiv = Jref*alpha + cross(w,Jref*w);
end

function [rate, accel] = pointDerivatives(r, u, ud)
rate = cross(u,r);
accel = cross(ud,r) + cross(u,rate);
end

function I = rodTensor(m, delta)
I = (m/12)*(dot(delta,delta)*eye(3) - delta*delta.');
end

function S = skew(v)
S = [0 -v(3) v(2); v(3) 0 -v(1); -v(2) v(1) 0];
end

== matlab function TVC_Hover_Plant_Coaxial_Articulated/TVC Plant/Weight in Body Axes ==
  data: C_BE input; F_g_B output; m input; g input
function F_g_B = body_weight(C_BE, m, g)
%#codegen
% NED gravity is +Z. Column 3 of C_BE is +Z_NED in body axes.
F_g_B = (m*g) * C_BE(:,3);
end

== matlab function TVC_Hover_Plant_Coaxial_Articulated/TVC Plant/TVC Kinematics ==
  data: T1 input; F_T_B output; T2 input; outer_deg input; inner_deg input; pivot input; link1 input; link2 input; kq1 input; kq2 input; M_B output; r_B output; r_inner_B output; axis_B output; Q output; thrust_N output; fan_y_B output
function [F_T_B, M_B, r_B, r_inner_B, axis_B, Q, thrust_N, fan_y_B] = tvc_kinematics(T1, T2, outer_deg, inner_deg, pivot, link1, link2, kq1, kq2)
%#codegen
% Angles rotate the links actively, following the right-hand rule.
a = outer_deg * (pi/180);
b = inner_deg * (pi/180);
ca = cos(a);
sa = sin(a);
cb = cos(b);
sb = sin(b);
R1 = [ca 0 sa; 0 1 0; -sa 0 ca];
R2 = [cb -sb 0; sb cb 0; 0 0 1];
R_motor = R1 * R2;
% Add both rotated link displacements to the fixed body-side pivot.
r_inner_B = pivot(:) + R1*link1(:);
r_B = r_inner_B + R_motor*link2(:);
axis_B = R_motor(:,1);
fan_y_B = R_motor(:,2);
thrust_N = [max(T1, 0); max(T2, 0)];
F_T_B = sum(thrust_N) * axis_B;
% Rotor spin signs are + and -. The reactions on the body are opposite.
Q = [-kq1*thrust_N(1); kq2*thrust_N(2)];
M_B = cross(r_B, F_T_B) + sum(Q)*axis_B;
end

== matlab function TVC_Hover_Plant_Coaxial_Articulated/TVC Plant/3D State ==
  data: pos input; frame output; C_BE input; pivot input; inner input; motor input; axis_B input; thrust input; fan_y_B input
function frame = flight_frame(pos, C_BE, pivot, inner, motor, axis_B, thrust, fan_y_B)
%#codegen
frame = [pos(:); C_BE(:); pivot(:); inner(:); motor(:); axis_B(:); thrust(:); fan_y_B(:)];
end

== matlab function TVC_Hover_Plant_Coaxial_Articulated/MATLAB Function1 ==
  settings: updateMethod=DISCRETE  sampleTime=0.01
  data: alpha_body input; T1_N output; T_total_N input; q_E_to_B input; omega_B input; T2_N output; outer_deg output; inner_deg output; TVC_INERTIA_KGM2 parameter double size=[3 3]; TVC_PIVOT_B_M parameter double size=[3 1]; TVC_LINK1_M parameter double size=[3 1]; TVC_LINK2_M parameter double size=[3 1]; TVC_FAN1_KQ parameter double size=[1 1]; TVC_FAN2_KQ parameter double size=[1 1]; TVC_TMAX1_N parameter double size=[1 1]; TVC_TMAX2_N parameter double size=[1 1]; TVC_SERVO_MAX_DEG parameter double size=[1 1]
function [T1_N, T2_N, outer_deg, inner_deg] = allocate_manual( ...
    alpha_body, T_total_N, q_E_to_B, omega_B, ...
    TVC_INERTIA_KGM2, TVC_PIVOT_B_M, TVC_LINK1_M, ...
    TVC_LINK2_M, TVC_FAN1_KQ, TVC_FAN2_KQ, ...
    TVC_TMAX1_N, TVC_TMAX2_N, TVC_SERVO_MAX_DEG)
%#codegen

% TVC Plant와 같은 값으로 설정
J = TVC_INERTIA_KGM2;
Jinv = J \ eye(3);

pivot = TVC_PIVOT_B_M;
link1 = TVC_LINK1_M;
link2 = TVC_LINK2_M;

kq1 = TVC_FAN1_KQ;
kq2 = TVC_FAN2_KQ;
Tmax1 = TVC_TMAX1_N;                % 팬 1 최대 추력 예시 [N]
Tmax2 = TVC_TMAX2_N;                % 팬 2 최대 추력 예시 [N]
servo_max = TVC_SERVO_MAX_DEG * (pi/180);      % 서보 제한 [rad]

Kp_roll = 13.5;
Kd_roll = 8.1;

% 조종기가 정한 총추력을 팬의 물리적 범위 안으로 제한
T = min(max(T_total_N, 0), Tmax1 + Tmax2);
T1_N = 0;
T2_N = 0;
outer_deg = 0;
inner_deg = 0;
if T <= 0
    return;
end

% 직립 자세를 기준으로 body +X축 비틀림 각도 추출
% 직립 자세의 Euler pitch가 90도이므로 쿼터니언으로 계산
c = sqrt(2)/2;
q_base_conj = [c; 0; -c; 0];
q = q_E_to_B(:);
q_norm = norm(q);

roll_rad = 0;
if isfinite(q_norm) && q_norm > 1e-12
    q_rel = quat_mul(q_base_conj, q/q_norm);
    if hypot(q_rel(1), q_rel(2)) > 1e-9
        roll_rad = 2*atan2(q_rel(2), q_rel(1));
        roll_rad = atan2(sin(roll_rad), cos(roll_rad));
    end
end

omega = omega_B(:);
alpha_cmd = alpha_body(:);
alpha_cmd(1) = -Kp_roll*roll_rad - Kd_roll*omega(1);

% 각속도 결합항을 보상한 목표 토크를 각가속도 단위로 표현
alpha_req = alpha_cmd + Jinv*cross(omega, J*omega);

% T1 + T2 = T 를 만족하는 팬 1의 추력 범위
T1_lo = max(0, T - Tmax2);
T1_hi = min(Tmax1, T);

best_a = 0;
best_b = 0;
best_cost = inf;
step = servo_max/4;

% 총추력을 고정한 상태에서 서보 각과 팬 추력차를 배분
for stage = 1:8
    center_a = best_a;
    center_b = best_b;
    radius = 1;
    if stage == 1
        radius = 4;
    end

    for i = -radius:radius
        a = min(max(center_a + i*step, -servo_max), servo_max);
        Ry = [cos(a) 0 sin(a); 0 1 0; -sin(a) 0 cos(a)];

        for j = -radius:radius
            b = min(max(center_b + j*step, -servo_max), servo_max);
            Rz = [cos(b) -sin(b) 0; sin(b) cos(b) 0; 0 0 1];

            R = Ry*Rz;
            d = R(:,1);
            r = pivot + Ry*link1 + R*link2;

            % 짐벌 토크와 팬 반작용 토크의 효과
            alpha_tvc = Jinv*cross(r, T*d);
            q_gain = Jinv*d;
            Q_req = dot(q_gain, alpha_req - alpha_tvc) / ...
                    dot(q_gain, q_gain);

            % Q = -kq1*T1 + kq2*T2, T1 + T2 = T
            if kq1 + kq2 > 0
                t1 = (kq2*T - Q_req)/(kq1 + kq2);
            else
                t1 = T/2;
            end
            t1 = min(max(t1, T1_lo), T1_hi);
            t2 = T - t1;

            Q = -kq1*t1 + kq2*t2;
            error = alpha_tvc + q_gain*Q - alpha_req;
            cost = dot(error, error);

            if cost < best_cost
                best_cost = cost;
                best_a = a;
                best_b = b;
                T1_N = t1;
                T2_N = t2;
            end
        end
    end
    step = step/2;
end

outer_deg = best_a*180/pi;
inner_deg = best_b*180/pi;
end

function q = quat_mul(p, r)
q = [p(1)*r(1) - dot(p(2:4), r(2:4));
     p(1)*r(2:4) + r(1)*p(2:4) + cross(p(2:4), r(2:4))];
end

== matlab function TVC_Hover_Plant_Coaxial_Articulated/MATLAB Function ==
  data: t input; T_total_N output
function T_total_N = throttle_profile(t)
%#codegen
% t: Clock 블록에서 들어오는 시뮬레이션 시간 [s]

T_peak = 8;     % 최대 총추력 [N]
t_up   = 1;     % 올라가는 시간 [s]
t_hold = 4.0;     % 유지 시간 [s]
t_down = 60.0;     % 내려가는 시간 [s]

hold_end = t_up + t_hold;
stop_time = hold_end + t_down;

if t < t_up
    T_total_N = T_peak * max(0, t/t_up);
elseif t < hold_end
    T_total_N = T_peak;
elseif t < stop_time
    T_total_N = T_peak * (stop_time - t)/t_down;
else
    T_total_N = 0;
end
end
